simulink model "CHB_Rectifier_LLC_Isolation"  (R2023b)
settings: Solver=VariableStepAuto  StartTime=0.0  StopTime=0.5  RelTol=1e-3
libraries: spsSeriesRLCBranchLib x8, spsVoltageMeasurementLib x7, spsUniversalBridgeLib x6, spsCurrentMeasurementLib x4, spsLinearTransformerLib x2, spsACVoltageSourceLib x1, simulink x1, spsMeanLib x1, spsMosfetLib x1, slpidlib x1, powerlib_extras x1, spsRMSLib x1
settings Model: SimulationMode=accelerator  Creator=Administrator  LastModifiedBy=Epiphanye

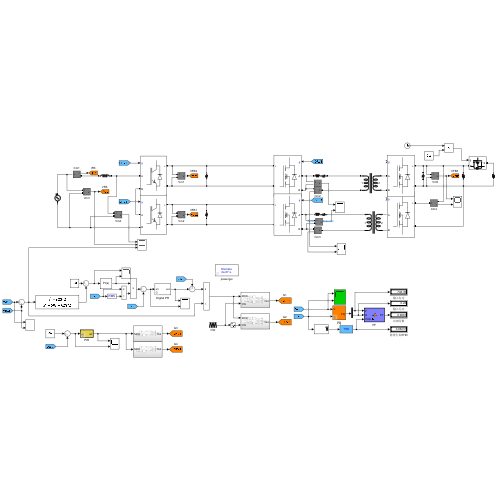
[thumbnail: Simulink's stored preview of the top-level diagram]
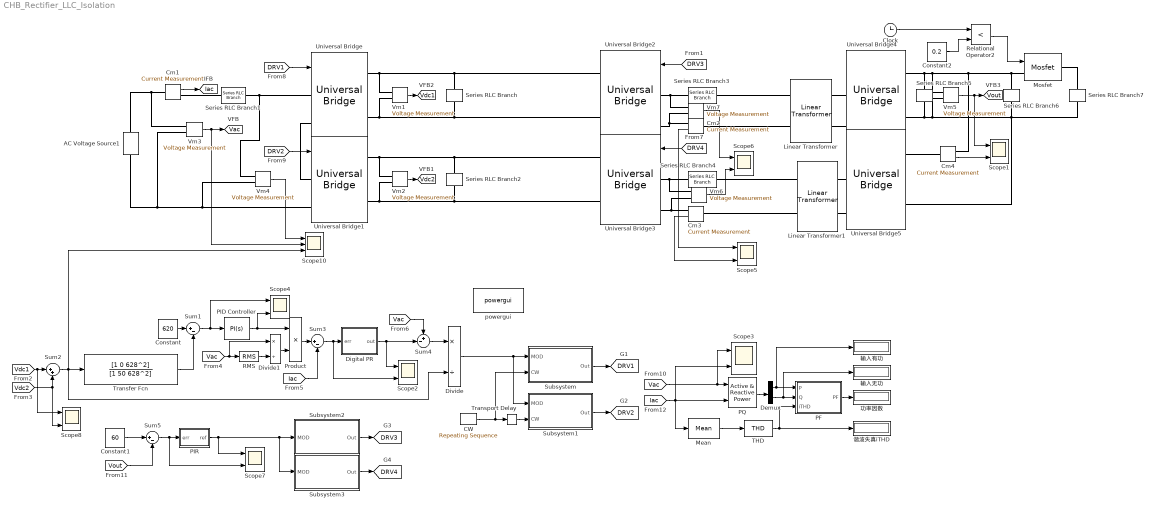
== system CHB_Rectifier_LLC_Isolation ==
  AC Voltage Source1 : spsACVoltageSourceLib/AC Voltage Source  Amplitude=537  Phase=0  Frequency=50  SampleTime=0  Measurements=None  BusType=swing  Pref=10e3  Qref=0  Qmin=-inf  Qmax=+inf
  CW : simulink/Sources/Repeating Sequence  rep_seq_t=[0 1/20000 1/10000]  rep_seq_y=[0 2 0]
  Clock : Clock
  Cm{1..4} (4 alike) : spsCurrentMeasurementLib/Current Measurement  PhasorSimulation=off  OutputType=Complex  PSBequivalent=0
  Constant : Constant  Value=620  VectorParams1D=off
  Constant1 : Constant  Value=60  VectorParams1D=off
  Constant2 : Constant  Value=0.2  VectorParams1D=off
  Demux : Demux  Outputs=2
  Digital PR : Subsystem  mask{Kp=8, Kr=100, Wc=5, Ts=1/40000, Upper=400, Lower=-400}
      mask DialogControl ParameterGroupVar Prompt: 参数
  Divide : Product  Inputs=*/
  Divide1 : Product  Inputs=*/
  Linear Transformer : spsLinearTransformerLib/Linear Transformer  UNITS=SI  NominalPower=[2500 60000]  winding1=[300 0.01 1e-6]  winding2=[100 0.01 1e-6]  ThreeWindings=off  winding3=[300 0.01 1e-6]  RmLm=[1e6 2e-4]  Measurements=None  DataType=on
  Linear Transformer1 : spsLinearTransformerLib/Linear Transformer  UNITS=SI  NominalPower=[2500 60000]  winding1=[300 0.01 1e-6]  winding2=[100 0.01 1e-6]  ThreeWindings=off  winding3=[300 0.01 1e-6]  RmLm=[1e6 2e-4]  Measurements=None  DataType=on
  Mean : spsMeanLib/Mean  Freq=10000  Vinit=0  Ts=0
  Mosfet : spsMosfetLib/Mosfet  Ron=0.01  Lon=0  Rd=0.01  Vfd=0  IC=0  Rs=1e5  Cs=inf  Measurements=off
  PF : MATLAB Function  TreatAsAtomicUnit=on
  PID Controller : slpidlib/PID Controller  Controller=PI  Form=Parallel  TimeDomain=Continuous-time  UseExternalTs=off  SampleTime=-1  IntegratorMethod=Forward Euler  FilterMethod=Forward Euler  ControllerParametersSource=internal  P=0.3  I=20  UseKiTs=off  D=0  N=100  UseFilter=on  TunerSelectOption=Transfer Function Based (PID Tuner App)  InitialConditionSource=internal  InitialConditionForIntegrator=0  InitialConditionForFilter=0  DifferentiatorICPrevScaledInput=0  ExternalReset=none  TrackingMode=off  Kt=1  LimitOutput=off  SatLimitsSource=internal  UpperSaturationLimit=50  LowerSaturationLimit=0  LinearizeAsGain=on  AntiWindupMode=none  Kb=1  LimitIntegrator=off  UpperIntegratorSaturationLimit=inf  LowerIntegratorSaturationLimit=-inf  POutMin=[]  POutMax=[]  IOutMin=[]  IOutMax=[]  DOutMin=[]  DOutMax=[]  NOutMin=[]  NOutMax=[]  SumOutMin=[]  SumOutMax=[]  SaturationOutMin=[]  SaturationOutMax=[]  PParamMin=[]  PParamMax=[]  IParamMin=[]  IParamMax=[]  DParamMin=[]  DParamMax=[]  NParamMin=[]  NParamMax=[]  KbParamMin=[]  KbParamMax=[]  KtParamMin=[]  KtParamMax=[]  KbOutMin=[]  KbOutMax=[]  KtOutMin=[]  KtOutMax=[]  IntegratorOutMin=[]  IntegratorOutMax=[]  FilterOutMin=[]  FilterOutMax=[]  SumI1OutMin=[]  SumI1OutMax=[]  SumI2OutMin=[]  SumI2OutMax=[]  SumI3OutMin=[]  SumI3OutMax=[]  SumI4OutMin=[]  SumI4OutMax=[]  SumDOutMin=[]  SumDOutMax=[]  DifferentiatorOutMin=[]  DifferentiatorOutMax=[]  FilterDiffOutCoefMin=[]  FilterDiffOutCoefMax=[]  ReciprocalOutMin=[]  ReciprocalOutMax=[]  SumDenOutMin=[]  SumDenOutMax=[]  SumNumOutMin=[]  SumNumOutMax=[]  DivideOutMin=[]  DivideOutMax=[]  UdiffTsProdOutMin=[]  UdiffTsProdOutMax=[]  NTsProdOutMin=[]  NTsProdOutMax=[]  UintegralTsProdOutMin=[]  UintegralTsProdOutMax=[]  UngainTsProdOutMin=[]  UngainTsProdOutMax=[]  ClampingZeroOutDataTypeStr=Inherit: Inherit via back propagation  ClampingZeroOutMin=[]  ClampingZeroOutMax=[]  FilterDenConstantOutDataTypeStr=Inherit: Inherit via back propagation  FilterDenConstantOutMin=[]  FilterDenConstantOutMax=[]  PCopyOutDataTypeStr=Inherit: Inherit via back propagation  PCopyOutMin=[]  PCopyOutMax=[]  NCopyOutDataTypeStr=Inherit: Inherit via back propagation  NCopyOutMin=[]  NCopyOutMax=[]  IntegratorContinuousStateAttributes=''  IntegratorStateMustResolveToSignalObject=off  IntegratorRTWStateStorageClass=Auto  FilterContinuousStateAttributes=''  FilterStateMustResolveToSignalObject=off  FilterRTWStateStorageClass=Auto  ParallelPVariant=InternalParameters  IdealPVariant=Disabled  IVariant=InternalParameters  DVariant=Disabled  IntegratorVariant=Continuous  SatVariant=Disabled  AWVariant=Passthrough  PCopyVariant=Disabled  TRVariant=Disabled  FdbkBlocksVariant=Forward  IdealPFdbkVariant=Disabled  SatFdbkVariant=Disabled  DerivativeFilterVariant=Disabled  NVariant=Disabled  NCopyVariant=Disabled_SignalSpec  FilterICVariant=Disabled  IntegratorICVariant=InternalICs  ExternalResetVariant=Disabled  TRSumVariant=Passthrough  SumFdbkVariant=Disabled  SumVariant=Sum_PI  TsampFilterVariant=InternalTs  TsampNgainVariant=Passthrough  TsampIntegralVariant=Disabled_SignalSpec  ExternalSaturationOutDataTypeStr=Inherit: Same as second input
  PIR : Subsystem  TreatAsAtomicUnit=on  mask{Kp=0.1, Kr=20, Wc=5, Upper=1, Lower=0}
  PQ : powerlib_extras/Measurements/Active & Reactive Power  f1=50
  Product : Product
  RMS : spsRMSLib/RMS  TrueRMS=on  Freq=50  RMSInit=380  Ts=0
  Relational Operator2 : RelationalOperator  Operator=<  OutDataTypeStr=boolean  InputSameDT=off
  Scope{1..8} (8 alike) : Scope  NumInputPorts=2
  Scope10 : Scope  NumInputPorts=3
  Series RLC Branch : spsSeriesRLCBranchLib/Series RLC Branch  LConnTagsString=__new0  RConnTagsString=__new0  BranchType=C  Resistance=0.1  Inductance=1e-3  SetiL0=off  InitialCurrent=0  Capacitance=2e-3  Setx0=on  InitialVoltage=300  Measurements=None
  Series RLC Branch1 : spsSeriesRLCBranchLib/Series RLC Branch  LConnTagsString=__new0  RConnTagsString=__new0  BranchType=L  Resistance=0.01  Inductance=3e-4  SetiL0=off  InitialCurrent=0  Capacitance=150e-6  Setx0=on  InitialVoltage=280  Measurements=None
  Series RLC Branch2 : spsSeriesRLCBranchLib/Series RLC Branch  LConnTagsString=__new0  RConnTagsString=__new0  BranchType=C  Resistance=0.1  Inductance=1e-3  SetiL0=off  InitialCurrent=0  Capacitance=2e-3  Setx0=on  InitialVoltage=280  Measurements=None
  Series RLC Branch3 : spsSeriesRLCBranchLib/Series RLC Branch  LConnTagsString=__new0  RConnTagsString=__new0  BranchType=LC  Resistance=0.1  Inductance=3e-5  SetiL0=off  InitialCurrent=0  Capacitance=2e-7  Setx0=off  InitialVoltage=155  Measurements=None
  Series RLC Branch4 : spsSeriesRLCBranchLib/Series RLC Branch  LConnTagsString=__new0  RConnTagsString=__new0  BranchType=LC  Resistance=0.1  Inductance=3e-5  SetiL0=off  InitialCurrent=0  Capacitance=2e-7  Setx0=off  InitialVoltage=155  Measurements=None
  Series RLC Branch5 : spsSeriesRLCBranchLib/Series RLC Branch  LConnTagsString=__new0  RConnTagsString=__new0  BranchType=C  Resistance=0.1  Inductance=1e-3  SetiL0=off  InitialCurrent=0  Capacitance=2e-3  Setx0=off  InitialVoltage=155  Measurements=None
  Series RLC Branch6 : spsSeriesRLCBranchLib/Series RLC Branch  LConnTagsString=__new0  RConnTagsString=__new0  BranchType=R  Resistance=5  Inductance=1e-3  SetiL0=off  InitialCurrent=0  Capacitance=2e-3  Setx0=on  InitialVoltage=155  Measurements=None
  Series RLC Branch7 : spsSeriesRLCBranchLib/Series RLC Branch  LConnTagsString=__new0  RConnTagsString=__new0  BranchType=R  Resistance=0.5  Inductance=1e-3  SetiL0=off  InitialCurrent=0  Capacitance=2e-3  Setx0=on  InitialVoltage=155  Measurements=None
  Subsystem : Subsystem
  Subsystem1 : Subsystem
  Subsystem2 : Subsystem
  Subsystem3 : Subsystem
  Sum1 : Sum  Inputs=|+-
  Sum2 : Sum  Inputs=|++
  Sum3 : Sum  Inputs=|+-
  Sum4 : Sum  Inputs=+-|
  Sum5 : Sum  Inputs=|+-
  THD : spsTHDLib/THD  Freq=50  Ts=0
  Transfer Fcn : TransferFcn  Numerator=[1 0 628^2]  Denominator=[1 50 628^2]
  Transport Delay : TransportDelay  DelayTime=1/10000/4
  Universal Bridge : spsUniversalBridgeLib/Universal Bridge  Arms=2  SnubberResistance=1e5  SnubberCapacitance=inf  Device=IGBT / Diodes  Ron=1e-3  Lon=0  ForwardVoltages="[  1  1  ]"  ForwardVoltage=0  GTOparameters=[ 10e-6 , 20e-6 ]  IGBTparameters=[ 1e-6 , 2e-6 ]  Measurements=None  Measurements_2=None  converterType=Rectifier
  Universal Bridge1 : spsUniversalBridgeLib/Universal Bridge  Arms=2  SnubberResistance=1e5  SnubberCapacitance=inf  Device=IGBT / Diodes  Ron=1e-3  Lon=0  ForwardVoltages="[  1  1  ]"  ForwardVoltage=0  GTOparameters=[ 10e-6 , 20e-6 ]  IGBTparameters=[ 1e-6 , 2e-6 ]  Measurements=None  Measurements_2=None  converterType=Rectifier
  Universal Bridge{2..5} (4 alike) : spsUniversalBridgeLib/Universal Bridge  Arms=2  SnubberResistance=1e5  SnubberCapacitance=inf  Device=MOSFET / Diodes  Ron=1e-3  Lon=0  ForwardVoltages="[  1  1  ]"  ForwardVoltage=0  GTOparameters=[ 10e-6 , 20e-6 ]  IGBTparameters=[ 1e-6 , 2e-6 ]  Measurements=None  Measurements_2=None  converterType=Rectifier
  Vm{1..7} (7 alike) : spsVoltageMeasurementLib/Voltage Measurement  PhasorSimulation=off  OutputType=Complex  PSBequivalent=0
  powergui : spspowerguiLib/powergui  Priority=1  SimulationMode=Discrete  SampleTime=2e-7  frequency=60  Iterations=50  frequencyindice=50  Pbase=100e6  ErrMax=1e-4  UnitsV=kV  UnitsW=MW  buscounter=0  FunctionMessages=off  echomessages=off  EnableUseOfTLC=off  CurrentSourceSwitches=off  DisableSnubberDevices=off  DisableRonSwitches=off  DisableVfSwitches=off  DisplayEquations=off  AutomaticDiscreteSolvers=off  SolverType=Tustin/Backward Euler (TBE)  Interpol=off  ExternalGateDelay=off  methode=off  Ts=100  x0status=blocks  SPID=on  SwTol=0  HookPort=off  NonlinearTolerance=1e-4  nMaxIteration=100  ContinueOnMaxIteration=off  RestoreLinks=warning  ResistiveCurrentMeasurement=off  Frange=[0:2:500]  Ylog=off  Xlog=on  ShowGrid=off  save=off  variable=ZData  structure=0  ZoomFFT=off  StartTime=0.0  cycles=1  DisplayStyle=1  fundamental=60  FreqAxis=off  MaxFrequency=1000  frequencyindicesteady=1  RmsSteady=1  display=off
  功率因数 : Display
  谐波失真iTHD : Display
  输入无功 : Display
      settings: Format=bank
  输入有功 : Display
      settings: Format=bank
  tag scope: DRV1=global, DRV2=global, DRV3=global, DRV4=global, Iac=global, Vac=global, Vdc1=global, Vdc2=global, Vout=global
  wires:
  Cm1/1 -> [Iac]
  Vm3/1 -> Scope10/2, [Vac]
  Vm1/1 -> [Vdc1]
  [Vdc1] -> Scope8/1, Sum2/1
  [Vdc2] -> Scope8/2, Sum2/2
  Sum1/1 -> PID Controller/1, Scope4/1
  Constant/1 -> Sum1/1
  PID Controller/1 -> Product/1, Scope4/2
  Product/1 -> Sum3/1
  [Iac] -> Sum3/2
  Sum2/1 -> Scope10/3, Divide/2, Transfer Fcn/1
  Divide/1 -> Subsystem1/1(MOD), Subsystem/1(MOD)
  CW/1 -> Subsystem/2(CW), Transport Delay/1
  Subsystem/1(Out) -> [DRV1]
  Subsystem1/1(Out) -> [DRV2]
  Transport Delay/1 -> Subsystem1/2(CW)
  [DRV1] -> Universal Bridge/1
  Transfer Fcn/1 -> Sum1/2
  PQ/1 -> Demux/1
  Demux/2 -> 输入无功/1, PF/2(Q)
  PF/1(PF) -> 功率因数/1
  THD/1 -> 谐波失真iTHD/1, PF/3(iTHD)
  Demux/1 -> 输入有功/1, PF/1(P)
  [Vac] -> Scope3/1, PQ/1
  [Iac] -> PQ/2, Scope3/2, Mean/1
  Mean/1 -> THD/1
  Vm2/1 -> [Vdc2]
  [DRV2] -> Universal Bridge1/1
  Vm4/1 -> Scope10/1
  Sum4/1 -> Divide/1
  [Vac] -> Sum4/1
  Sum3/1 -> Scope2/2, Digital PR/1(err)
  Digital PR/1(out) -> Scope2/1, Sum4/2
  Divide1/1 -> Product/2
  RMS/1 -> Divide1/2
  [Vac] -> Divide1/1, RMS/1
  Vm5/1 -> [Vout], Scope1/1
  Cm4/1 -> Scope1/2
  Cm3/1 -> Scope5/2
  Cm2/1 -> Scope5/1
  Subsystem2/1(Out) -> [DRV3]
  Subsystem3/1(Out) -> [DRV4]
  Vm7/1 -> Scope6/1
  Vm6/1 -> Scope6/2
  [DRV3] -> Universal Bridge2/1
  [DRV4] -> Universal Bridge3/1
  Constant1/1 -> Sum5/1
  [Vout] -> Sum5/2
  Sum5/1 -> Scope7/2, PIR/1(err)
  PIR/1(ref) -> Scope7/1, Subsystem3/1(MOD), Subsystem2/1(MOD)
  Clock/1 -> Relational Operator2/1
  Constant2/1 -> Relational Operator2/2
  Relational Operator2/1 -> Mosfet/1
  connections:
  Universal Bridge/RConn2 -- Series RLC Branch/RConn1 -- Universal Bridge2/RConn2 -- Vm1/LConn2
  Vm1/LConn1 -- Universal Bridge2/RConn1 -- Series RLC Branch/LConn1 -- Universal Bridge/RConn1
  Cm1/LConn1 -- AC Voltage Source1/RConn1 -- Vm3/LConn1
  AC Voltage Source1/LConn1 -- Vm4/LConn2 -- Universal Bridge1/LConn2 -- Vm3/LConn2
  Series RLC Branch1/LConn1 -- Cm1/RConn1
  Universal Bridge/LConn1 -- Vm4/LConn1 -- Series RLC Branch1/RConn1
  Series RLC Branch2/RConn1 -- Vm2/LConn2 -- Universal Bridge1/RConn2 -- Universal Bridge3/RConn2
  Series RLC Branch2/LConn1 -- Vm2/LConn1 -- Universal Bridge1/RConn1 -- Universal Bridge3/RConn1
  Universal Bridge/LConn2 -- Universal Bridge1/LConn1
  Series RLC Branch3/LConn1 -- Vm7/LConn1 -- Universal Bridge2/LConn1
  Series RLC Branch4/LConn1 -- Vm6/LConn1 -- Universal Bridge3/LConn1
  Cm2/RConn1 -- Vm7/LConn2 -- Universal Bridge2/LConn2
  Cm3/RConn1 -- Vm6/LConn2 -- Universal Bridge3/LConn2
  Linear Transformer/LConn1 -- Series RLC Branch3/RConn1
  Linear Transformer/LConn2 -- Cm2/LConn1
  Linear Transformer1/LConn1 -- Series RLC Branch4/RConn1
  Linear Transformer1/LConn2 -- Cm3/LConn1
  Universal Bridge4/LConn1 -- Linear Transformer/RConn1
  Universal Bridge4/LConn2 -- Linear Transformer/RConn2
  Universal Bridge5/LConn1 -- Linear Transformer1/RConn1
  Universal Bridge5/LConn2 -- Linear Transformer1/RConn2
  Series RLC Branch5/LConn1 -- Series RLC Branch6/LConn1 -- Mosfet/LConn1 -- Cm4/RConn1 -- Vm5/LConn1 -- Universal Bridge4/RConn1
  Universal Bridge5/RConn2 -- Series RLC Branch6/RConn1 -- Series RLC Branch7/RConn1 -- Universal Bridge4/RConn2 -- Series RLC Branch5/RConn1 -- Vm5/LConn2
  Cm4/LConn1 -- Universal Bridge5/RConn1
  Mosfet/RConn1 -- Series RLC Branch7/LConn1

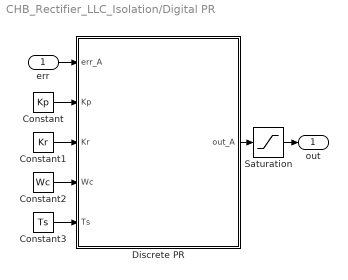
== system CHB_Rectifier_LLC_Isolation/Digital PR ==
  err : Inport
  Constant : Constant  Value=Kp
  Constant1 : Constant  Value=Kr
  Constant2 : Constant  Value=Wc
  Constant3 : Constant  Value=Ts
  Discrete PR : MATLAB Function  TreatAsAtomicUnit=on
  Saturation : Saturate  UpperLimit=Upper  LowerLimit=Lower
  out : Outport
  wires:
  Constant1/1 -> Discrete PR/3(Kr)
  Constant3/1 -> Discrete PR/5(Ts)
  Constant/1 -> Discrete PR/2(Kp)
  Constant2/1 -> Discrete PR/4(Wc)
  Discrete PR/1(out_A) -> Saturation/1
  Saturation/1 -> out/1
  err/1 -> Discrete PR/1(err_A)

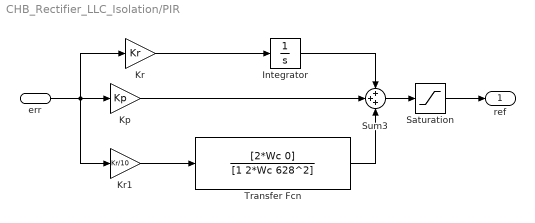
== system CHB_Rectifier_LLC_Isolation/PIR ==
  err : Inport
  Integrator : Integrator
  Kp : Gain  Gain=Kp
  Kr : Gain  Gain=Kr
  Kr1 : Gain  Gain=Kr/10
  Saturation : Saturate  UpperLimit=Upper  LowerLimit=Lower
  Sum3 : Sum  Inputs=+++
  Transfer Fcn : TransferFcn  Numerator=[2*Wc 0]  Denominator=[1 2*Wc 628^2]
  ref : Outport
  wires:
  Sum3/1 -> Saturation/1
  err/1 -> Kr1/1, Kr/1, Kp/1
  Saturation/1 -> ref/1
  Kp/1 -> Sum3/2
  Transfer Fcn/1 -> Sum3/3
  Integrator/1 -> Sum3/1
  Kr/1 -> Integrator/1
  Kr1/1 -> Transfer Fcn/1

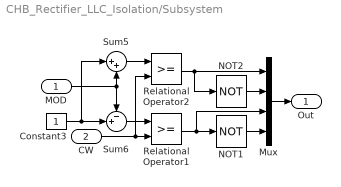
== system CHB_Rectifier_LLC_Isolation/Subsystem ==
  MOD : Inport
  CW : Inport  Port=2
  Constant3 : Constant  VectorParams1D=off
  Mux : Mux
  NOT1 : Logic  Operator=NOT  IconShape=distinctive  AllPortsSameDT=off  OutDataTypeStr=boolean
  NOT2 : Logic  Operator=NOT  IconShape=distinctive  AllPortsSameDT=off  OutDataTypeStr=boolean
  Relational Operator1 : RelationalOperator  OutDataTypeStr=boolean  InputSameDT=off
  Relational Operator2 : RelationalOperator  OutDataTypeStr=boolean  InputSameDT=off
  Sum5 : Sum  Inputs=|++
  Sum6 : Sum  Inputs=-+|
  Out : Outport
  wires:
  Sum6/1 -> Relational Operator1/1
  Constant3/1 -> Sum5/1, Sum6/2
  MOD/1 -> Sum6/1, Sum5/2
  CW/1 -> Relational Operator2/2, Relational Operator1/2
  Relational Operator2/1 -> Mux/1, NOT2/1
  Sum5/1 -> Relational Operator2/1
  NOT1/1 -> Mux/4
  Relational Operator1/1 -> Mux/3, NOT1/1
  NOT2/1 -> Mux/2
  Mux/1 -> Out/1

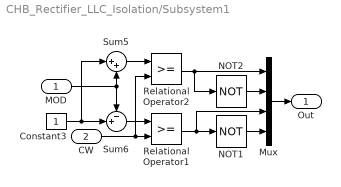
== system CHB_Rectifier_LLC_Isolation/Subsystem1 ==
  MOD : Inport
  CW : Inport  Port=2
  Constant3 : Constant  VectorParams1D=off
  Mux : Mux
  NOT1 : Logic  Operator=NOT  IconShape=distinctive  AllPortsSameDT=off  OutDataTypeStr=boolean
  NOT2 : Logic  Operator=NOT  IconShape=distinctive  AllPortsSameDT=off  OutDataTypeStr=boolean
  Relational Operator1 : RelationalOperator  OutDataTypeStr=boolean  InputSameDT=off
  Relational Operator2 : RelationalOperator  OutDataTypeStr=boolean  InputSameDT=off
  Sum5 : Sum  Inputs=|++
  Sum6 : Sum  Inputs=-+|
  Out : Outport
  wires:
  Mux/1 -> Out/1
  NOT2/1 -> Mux/2
  Relational Operator1/1 -> NOT1/1, Mux/3
  NOT1/1 -> Mux/4
  Sum5/1 -> Relational Operator2/1
  Relational Operator2/1 -> NOT2/1, Mux/1
  CW/1 -> Relational Operator1/2, Relational Operator2/2
  MOD/1 -> Sum5/2, Sum6/1
  Constant3/1 -> Sum6/2, Sum5/1
  Sum6/1 -> Relational Operator1/1

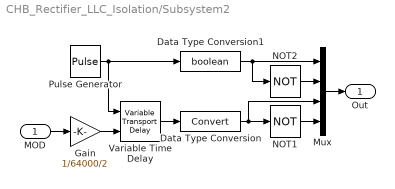
== system CHB_Rectifier_LLC_Isolation/Subsystem2 ==
  MOD : Inport
  Data Type Conversion : DataTypeConversion  SaturateOnIntegerOverflow=off  RndMeth=Floor
  Data Type Conversion1 : DataTypeConversion  OutDataTypeStr=boolean  SaturateOnIntegerOverflow=off  RndMeth=Floor
  Gain : Gain  Gain=1/64000/2
  Mux : Mux
  NOT1 : Logic  Operator=NOT  IconShape=distinctive  AllPortsSameDT=off  OutDataTypeStr=boolean
  NOT2 : Logic  Operator=NOT  IconShape=distinctive  AllPortsSameDT=off  OutDataTypeStr=boolean
  Pulse Generator : DiscretePulseGenerator  PulseType=Time based  Period=1/64000  PulseWidth=50
  Variable Time Delay : VariableTransportDelay  MaximumDelay=10
  Out : Outport
  wires:
  Mux/1 -> Out/1
  NOT2/1 -> Mux/2
  NOT1/1 -> Mux/4
  Pulse Generator/1 -> Data Type Conversion1/1, Variable Time Delay/1
  MOD/1 -> Gain/1
  Gain/1 -> Variable Time Delay/2
  Variable Time Delay/1 -> Data Type Conversion/1
  Data Type Conversion/1 -> Mux/3, NOT1/1
  Data Type Conversion1/1 -> NOT2/1, Mux/1

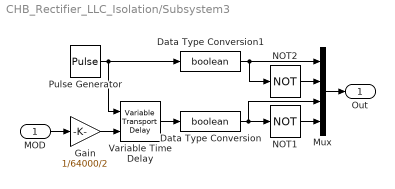
== system CHB_Rectifier_LLC_Isolation/Subsystem3 ==
  MOD : Inport
  Data Type Conversion : DataTypeConversion  OutDataTypeStr=boolean  SaturateOnIntegerOverflow=off  RndMeth=Floor
  Data Type Conversion1 : DataTypeConversion  OutDataTypeStr=boolean  SaturateOnIntegerOverflow=off  RndMeth=Floor
  Gain : Gain  Gain=1/64000/2
  Mux : Mux
  NOT1 : Logic  Operator=NOT  IconShape=distinctive  AllPortsSameDT=off  OutDataTypeStr=boolean
  NOT2 : Logic  Operator=NOT  IconShape=distinctive  AllPortsSameDT=off  OutDataTypeStr=boolean
  Pulse Generator : DiscretePulseGenerator  PulseType=Time based  Period=1/64000  PulseWidth=50  PhaseDelay=1/64000/4
  Variable Time Delay : VariableTransportDelay  MaximumDelay=10
  Out : Outport
  wires:
  Data Type Conversion/1 -> NOT1/1, Mux/3
  Variable Time Delay/1 -> Data Type Conversion/1
  Gain/1 -> Variable Time Delay/2
  MOD/1 -> Gain/1
  Pulse Generator/1 -> Data Type Conversion1/1, Variable Time Delay/1
  NOT1/1 -> Mux/4
  NOT2/1 -> Mux/2
  Mux/1 -> Out/1
  Data Type Conversion1/1 -> NOT2/1, Mux/1

== matlab function CHB_Rectifier_LLC_Isolation/PF ==
  data: P input; PF output; Q input; iTHD input
function PF = fcn(P,Q,iTHD)
% This block supports an embeddable subset of the MATLAB language.
% See the help menu for details. 
PF=(P/sqrt(P*P+Q*Q))/(sqrt(1+iTHD*iTHD));

== matlab function CHB_Rectifier_LLC_Isolation/Digital PR/Discrete PR ==
  settings: updateMethod=DISCRETE  sampleTime=Ts
  data: err_A input; out_A output; Kp input; Kr input; Wc input; Ts input
function out_A  = fcn(err_A, Kp, Kr, Wc, Ts)

W0 = 50*2*pi;


persistent err_A1;
persistent err_A2;
persistent out_A1;
persistent out_A2;


%%对三相静态变量初始化
if isempty(err_A1)
    err_A1 = 0;
end
if isempty(err_A2)
    err_A2 = 0;
end
if isempty(out_A1)
    out_A1 = 0;
end
if isempty(out_A2)
    out_A2 = 0;
end


%%Discrete
t1 = Wc * Ts;
t2 = W0^2 * Ts^2;
t3 = t2 + 4*t1 + 4;

b0 = (Kp*t2 + 4*(Kp+Kr)*t1 + 4*Kp) / t3;
b1 = (2*Kp*t2 - 8*Kp) / t3;
b2 = (Kp*t2 + 4*Kp - 4*(Kp+Kr)*t1) / t3;
a1 = (2*t2 - 8) / t3;
a2 = (t2 - 4*t1 + 4) / t3;
%%限制输出
if b0>3000
    b0=0;
end
if b0<-3000
    b0=0;
end

%%计算输出量
out_A = b0*err_A + b1*err_A1 + b2*err_A2 - a1*out_A1 - a2*out_A2;
out_A2 = out_A1;
out_A1 = out_A;
err_A2 = err_A1;
err_A1 = err_A;
